simulink model "limo_gazebo_R2026a"  (R2026a)
settings: Solver=ode15s  StopTime=10  RelTol=1e-6  AbsTol=1e-8
PostLoadFcn:
  | addpath(fileparts(get_param(bdroot, 'FileName')));
libraries: limo_lib x1
settings Model: Creator=jkreiss  LastModifiedBy=mattia
settings SFSimCC: SimGPUStackLimitPerThread=51200
settings RTWCC: GPUStackLimitPerThread=51200

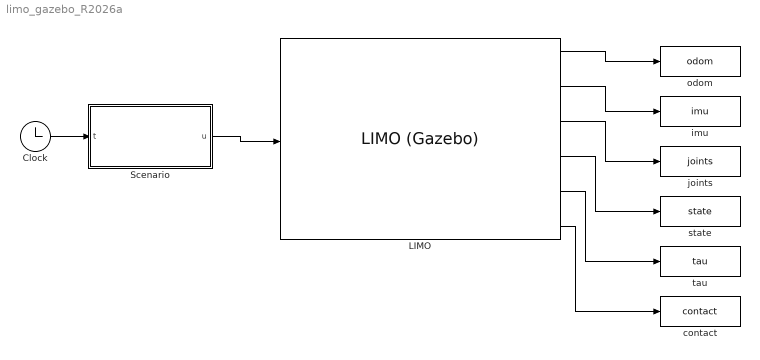
== system limo_gazebo_R2026a ==
  Clock : Clock
  LIMO : limo_lib/LIMO (Gazebo)  input_mode=Steering angle: [v; gamma]  pose_mode=Origin  custom_pose=[0 0 0]  mu=1  v_eps=1e-3
  Scenario : MATLAB Function  TreatAsAtomicUnit=on
  contact : ToWorkspace  VariableName=contact  SaveFormat=Timeseries  SampleTime=-1
  imu : ToWorkspace  VariableName=imu  SaveFormat=Timeseries  SampleTime=-1
  joints : ToWorkspace  VariableName=joints  SaveFormat=Timeseries  SampleTime=-1
  odom : ToWorkspace  VariableName=odom  SaveFormat=Timeseries  SampleTime=-1
  state : ToWorkspace  VariableName=state  SaveFormat=Timeseries  SampleTime=-1
  tau : ToWorkspace  VariableName=tau  SaveFormat=Timeseries  SampleTime=-1
  wires:
  Clock/1 -> Scenario/1(t)
  Scenario/1(u) -> LIMO/1
  LIMO/1 -> odom/1
  LIMO/2 -> imu/1
  LIMO/3 -> joints/1
  LIMO/4 -> state/1
  LIMO/5 -> tau/1
  LIMO/6 -> contact/1

== matlab function limo_gazebo_R2026a/Scenario ==
  data: t input; u output
function u = scenario(t)
%SCENARIO Speed and steering angle as a function of time.
%   u = [v (m/s); gamma (rad)], gamma > 0 to the left

v = 0;
gamma = 0;

if t >= 0.5
    v = 0.5;
end

if t >= 3 && t < 8
    gamma = 0.3;
end

u = [v; gamma];
